simulink model "pid_board_cl"  (R2024b)
settings: Solver=ode4  StartTime=0.0  StopTime=pbsim.t_stop  FixedStep=pcb.sim_dt  RelTol=1e-3
PostLoadFcn:
  | pbdir_ = fileparts(get_param('pid_board_cl', 'FileName')); if ~exist('pcb', 'var'), run(fullfile(pbdir_, 'pid_board_params.m')); end; if ~exist('CtrlIn', 'var'), run(fullfile(pbdir_, '..', 'common', 'quad_ctrl_buses.m')); end; clear pbdir_
undefined symbols (not defined in the file or in its folder): pbsim
settings Model: Creator=doubi  LastModifiedBy=doubi

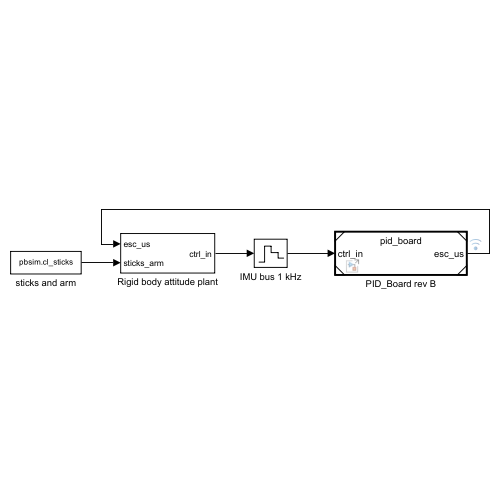
[thumbnail: Simulink's stored preview of the top-level diagram]
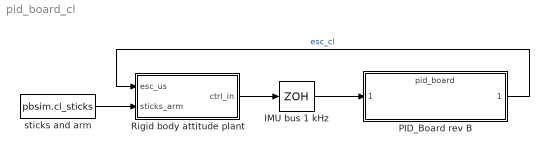
== system pid_board_cl ==
  IMU bus 1 kHz : ZeroOrderHold  SampleTime=1e-3
  PID_Board rev B : ModelReference  ModelNameDialog=pid_board  ParameterArgumentNames=board_variant  ParameterArgumentValues=pcb.variant  UsingDefaultArgumentValue=0  SimulationMode=Normal  ModelReferenceVersion=1.1
  Rigid body attitude plant : Subsystem  mask{pl=pbsim.plant}
  sticks and arm : FromWorkspace  VariableName=pbsim.cl_sticks  Interpolate=off  OutputAfterFinalValue=Holding final value
  wires:
  IMU bus 1 kHz/1 -> PID_Board rev B/1
  sticks and arm/1 -> Rigid body attitude plant/2(sticks_arm)
  PID_Board rev B/1 -> Rigid body attitude plant/1(esc_us)  "esc_cl"
  Rigid body attitude plant/1(ctrl_in) -> IMU bus 1 kHz/1

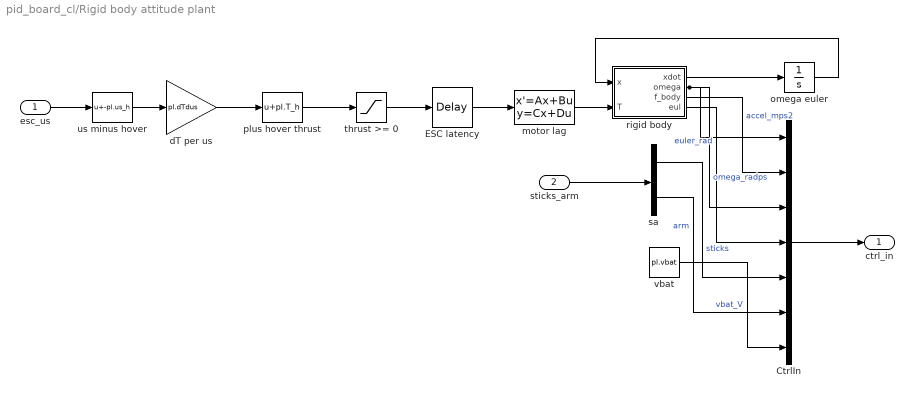
== system pid_board_cl/Rigid body attitude plant ==
  esc_us : Inport
  sticks_arm : Inport  Port=2
  CtrlIn : BusCreator  Inputs=7  OutDataTypeStr=Bus: CtrlIn
      settings: InheritFromInputs=off
  ESC latency : TransportDelay  DelayTime=pl.t_lat  InitialOutput=pl.T_h
  dT per us : Gain  Gain=pl.dTdus
  motor lag : StateSpace  A=-eye(4)/pl.tau  B=eye(4)/pl.tau  C=eye(4)  D=zeros(4)  InitialCondition=pl.T_h*ones(4,1)
  omega euler : Integrator  InitialCondition=pl.x0
  plus hover thrust : Bias  Bias=pl.T_h  SaturateOnIntegerOverflow=off
  rigid body : MATLAB Function  TreatAsAtomicUnit=on
  sa : Demux  Outputs=[4 1]
  thrust >= 0 : Saturate  UpperLimit=pl.T_max  LowerLimit=0
  us minus hover : Bias  Bias=-pl.us_h  SaturateOnIntegerOverflow=off
  vbat : Constant  Value=pl.vbat  SampleTime=0
  ctrl_in : Outport
  wires:
  plus hover thrust/1 -> thrust >= 0/1
  us minus hover/1 -> dT per us/1
  esc_us/1 -> us minus hover/1
  sticks_arm/1 -> sa/1
  thrust >= 0/1 -> ESC latency/1
  dT per us/1 -> plus hover thrust/1
  ESC latency/1 -> motor lag/1
  motor lag/1 -> rigid body/2(T)
  omega euler/1 -> rigid body/1(x)
  rigid body/1(xdot) -> omega euler/1
  rigid body/2(omega) -> CtrlIn/1, CtrlIn/3  "omega_radps"
  vbat/1 -> CtrlIn/7  "vbat_V"
  rigid body/3(f_body) -> CtrlIn/2  "accel_mps2"
  rigid body/4(eul) -> CtrlIn/4  "euler_rad"
  sa/1 -> CtrlIn/5  "sticks"
  sa/2 -> CtrlIn/6  "arm"
  CtrlIn/1 -> ctrl_in/1

== matlab function pid_board_cl/Rigid body attitude plant/rigid body ==
  data: x input size=[6 1]; xdot output size=[6 1]; T input size=[4 1]; omega output size=[3 1]; f_body output size=[3 1]; eul output size=[3 1]; pl parameter
function [xdot, omega, f_body, eul] = rb(x, T, pl)
%Rigid-body attitude dynamics (FRD), thrust T(4) along -z at r_i, Q_i = -spin_i*kQ/kT*T_i
omega = x(1:3); eul = x(4:6);
tau = [-pl.ry*T; pl.rx*T; -(pl.spin*T)*pl.kQT];
wdot = pl.Jinv*(tau - cross(omega, pl.J*omega) - pl.krot.*omega);
ph = eul(1); th = eul(2);
p = omega(1); q = omega(2); r = omega(3);
eulDot = [p + (q*sin(ph) + r*cos(ph))*tan(th); q*cos(ph) - r*sin(ph); (q*sin(ph) + r*cos(ph))/cos(th)];
xdot = [wdot; eulDot];
% quasi-static specific force (hover in place): -gravity in body axes
f_body = pl.g*[sin(th); -sin(ph)*cos(th); -cos(ph)*cos(th)];
